simulink model "Progetto_Hinf_simulink"  (R2026a)
settings: Solver=VariableStepAuto
InitFcn:
  | actuator = actuator_params_nominal();
  | [Gact, info] = build_nominal_actuator(actuator);
  | 
  | % Parametri del robot
  | p = sea_params_nominal();
  | Simulink.Bus.createObject(p);
  | 
  | % Equilibrio desiderato
  | qbar = [pi/2; 0];
  | 
  | % Calcolo stato e coppia di equilibrio
  | [xbar, taubar, info] = sea_static_equilibrium(qbar, p);
undefined symbols (not defined in the file): Ak, Bk, Ck, Dk, taubar, xbar
libraries: cstblocks_lti x2
settings Model: Creator=rebec  LastModifiedBy=rebec

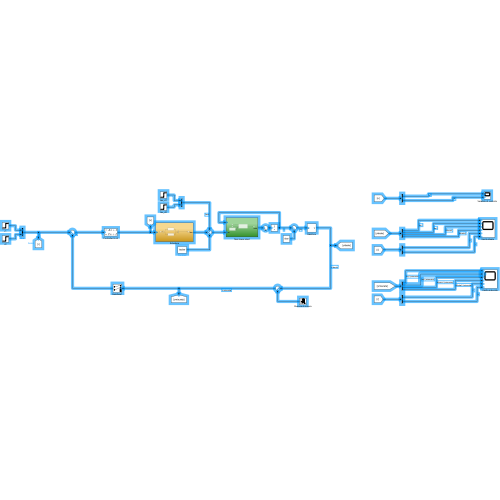
[thumbnail: Simulink's stored preview of the top-level diagram]
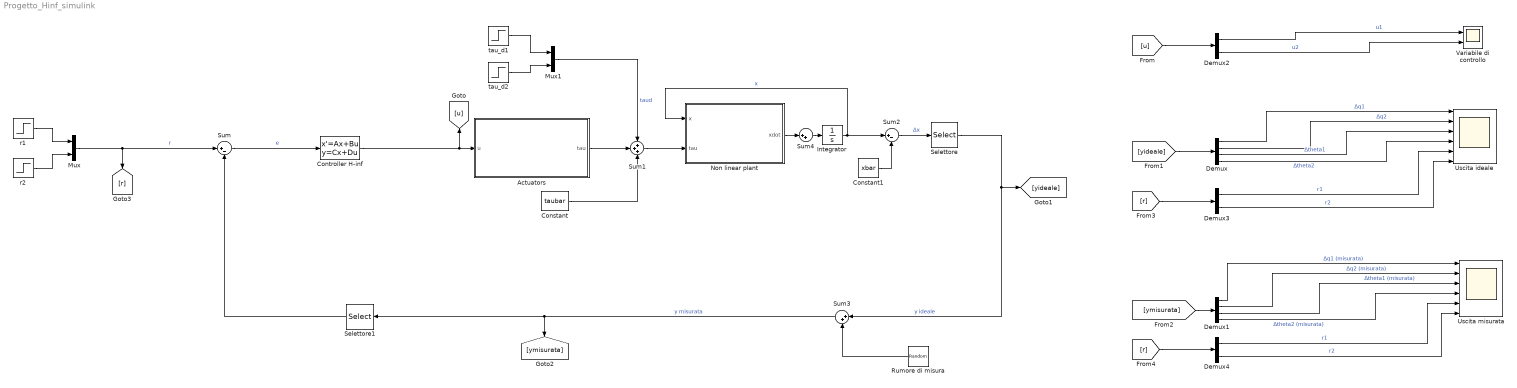
== system Progetto_Hinf_simulink ==
  Actuators : Subsystem
  Constant : Constant  Value=taubar
  Constant1 : Constant  Value=xbar
  Controller H-inf : StateSpace  A=Ak  B=Bk  C=Ck  D=Dk  InitialCondition=0
  Demux : Demux
  Demux1 : Demux
  Demux2 : Demux  Outputs=2
  Demux3 : Demux  Outputs=2
  Demux4 : Demux  Outputs=2
  Integrator : Integrator  InitialCondition=xbar
  Mux : Mux  Inputs=2
  Mux1 : Mux  Inputs=2
  Non linear plant : Subsystem
  Rumore di misura : RandomNumber  Variance=(0.05*pi/180)^2  Seed=20260826  SampleTime=0.002
  Selettore : Selector  InputPortWidth=8  IndexOptions=Index vector (dialog)  Indices=[1 2 5 6]  OutputSizes=1
  Selettore1 : Selector  InputPortWidth=4  IndexOptions=Index vector (dialog)  Indices=[1 2]  OutputSizes=1
  Sum : Sum  Inputs=|+-
  Sum1 : Sum  Inputs=+++
  Sum2 : Sum  Inputs=|+-
  Sum3 : Sum  Inputs=|++
  Sum4 : Sum  Inputs=|++
  Uscita ideale : Scope  NumInputPorts=6
      settings: Title=y (uscita ideale)  ActiveDisplayYMinimum=-0.6065472521807  ActiveDisplayYMaximum=0.64249935531189384
  Uscita misurata : Scope  NumInputPorts=6
      settings: Title=y (uscita ideale)  ActiveDisplayYMinimum=-0.54348624607883766  ActiveDisplayYMaximum=0.4563878411340912
  Variabile di controllo : Scope  NumInputPorts=2
      settings: ActiveDisplayYMinimum=-2.6959450601265313  ActiveDisplayYMaximum=5.9059369724787079  DataLoggingVariableName=ScopeData2
  r1 : Step  FinalValue=5*pi/180  SampleTime=0
  r2 : Step  FinalValue=0  SampleTime=0
  tau_d1 : Step  FinalValue=0.5  SampleTime=0
  tau_d2 : Step  FinalValue=0  SampleTime=0
  wires:
  Actuators/1(tau) -> Sum1/2
  tau_d1/1 -> Mux1/1
  tau_d2/1 -> Mux1/2
  Demux3/2 -> Uscita ideale/6  "r2"
  Demux4/1 -> Uscita misurata/5  "r1"
  Mux1/1 -> Sum1/1  "taud"
  [r] -> Demux4/1
  [r] -> Demux3/1
  Demux/4 -> Uscita ideale/4  "Δtheta2"
  Demux/1 -> Uscita ideale/1  "Δq1"
  Demux/3 -> Uscita ideale/3  "Δtheta1"
  Demux4/2 -> Uscita misurata/6  "r2"
  Sum4/1 -> Integrator/1
  Non linear plant/1(xdot) -> Sum4/1
  Constant/1 -> Sum1/3
  Demux1/1 -> Uscita misurata/1  "Δq1 (misurata)"
  [yideale] -> Demux/1
  Demux1/2 -> Uscita misurata/2  "Δq2 (misurata)"
  Demux1/4 -> Uscita misurata/4  "Δtheta2 (misurata)"
  Demux2/1 -> Variabile di controllo/1  "u1"
  Demux/2 -> Uscita ideale/2  "Δq2"
  [u] -> Demux2/1
  Rumore di misura/1 -> Sum3/2
  Mux/1 -> Sum/1, [r]  "r"
  [ymisurata] -> Demux1/1
  r1/1 -> Mux/1
  Selettore/1 -> [yideale], Sum3/1  "y ideale"
  Sum3/1 -> Selettore1/1, [ymisurata]  "y misurata"
  Integrator/1 -> Non linear plant/1(x), Sum2/1  "x"
  Demux2/2 -> Variabile di controllo/2  "u2"
  Demux3/1 -> Uscita ideale/5  "r1"
  Sum1/1 -> Non linear plant/2(tau)
  r2/1 -> Mux/2
  Demux1/3 -> Uscita misurata/3  "Δtheta1 (misurata)"
  Constant1/1 -> Sum2/2
  Sum2/1 -> Selettore/1  "Δx"
  Sum/1 -> Controller H-inf/1  "e"
  Controller H-inf/1 -> [u], Actuators/1(u)
  Selettore1/1 -> Sum/2

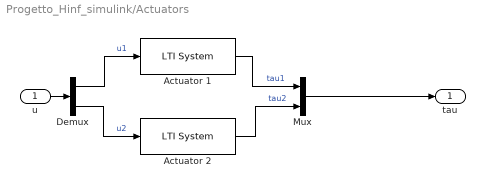
== system Progetto_Hinf_simulink/Actuators ==
  u : Inport
  Actuator 1 : cstblocks_lti/LTI System  sys=Gact  IC=[]  PadeOrder=0
      settings: LibrarySourceBlock=cstblocks/LTI System
  Actuator 2 : cstblocks_lti/LTI System  sys=Gact  IC=[]  PadeOrder=0
      settings: LibrarySourceBlock=cstblocks/LTI System
  Demux : Demux  Outputs=2
  Mux : Mux  Inputs=2
  tau : Outport
  wires:
  Actuator 2/1 -> Mux/2  "tau2"
  Demux/2 -> Actuator 2/1  "u2"
  u/1 -> Demux/1
  Demux/1 -> Actuator 1/1  "u1"
  Mux/1 -> tau/1
  Actuator 1/1 -> Mux/1  "tau1"

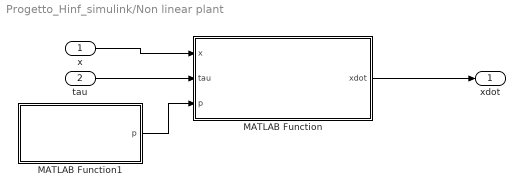
== system Progetto_Hinf_simulink/Non linear plant ==
  x : Inport
  tau : Inport  Port=2
  MATLAB Function : MATLAB Function  TreatAsAtomicUnit=on
  MATLAB Function1 : MATLAB Function  TreatAsAtomicUnit=on
  xdot : Outport
  wires:
  x/1 -> MATLAB Function/1(x)
  tau/1 -> MATLAB Function/2(tau)
  MATLAB Function/1(xdot) -> xdot/1
  MATLAB Function1/1(p) -> MATLAB Function/3(p)

== matlab function Progetto_Hinf_simulink/Non linear plant/MATLAB Function ==
  data: x input; xdot output; tau input; p input
function xdot = sea_nonlinear_rhs(x, tau, p)
%SEA_NONLINEAR_RHS Full eight-state nonlinear dynamics of the 2R SEA robot.
%   X = [q; qdot; theta; thetadot] is an 8-by-1 state vector and TAU is
%   the 2-by-1 motor torque in N*m. The output follows the same state order.

assert(numel(x) == 8, 'sea_nonlinear_rhs:InvalidState', ...
    'The state must contain exactly eight elements.');
assert(numel(tau) == 2, 'sea_nonlinear_rhs:InvalidInput', ...
    'The motor torque must contain exactly two elements.');

x = reshape(x, 8, 1);
tau = reshape(tau, 2, 1);

q = x(1:2);
qdot = x(3:4);
theta = x(5:6);
thetadot = x(7:8);

M = sea_link_inertia(q, p);
C = sea_coriolis(q, qdot, p);
G = sea_gravity(q, p);
tauElastic = sea_elastic_torque(q, theta, p);

qddot = M \ (tauElastic - C * qdot - G);
thetaddot = p.Jm \ (tau - p.Bm * thetadot - tauElastic);

xdot = [qdot; qddot; thetadot; thetaddot];
end

== matlab function Progetto_Hinf_simulink/Non linear plant/MATLAB Function1 ==
  data: p output Bus: slBus1
function p = sea_params_nominal
%SEA_PARAMS_NOMINAL Nominal mechanical parameters of the 2R SEA robot.
%   P = SEA_PARAMS_NOMINAL returns the values stated by the official
%   assignment. Matrices follow the joint order [joint 1; joint 2].

p.m1 = 1.0;                   % kg
p.m2 = 0.8;                   % kg
p.l1 = 0.4;                   % m
p.l2 = 0.3;                   % m
p.Jm = diag([0.01, 0.01]);    % kg*m^2
p.Bm = diag([0.02, 0.02]);    % N*m*s/rad
p.Ks = diag([50, 40]);        % N*m/rad
p.g = 9.81;                   % m/s^2
end
